simulink model "single_phase_cllc_param"  (R2026a)
settings: Solver=ode23tb  StopTime=param.sim.simlength  FixedStep=tc  MaxStep=param.glb_time.tc
values from neighbouring files (symbols this model uses):
  param = add_template_extras(param, options)    [init_model.m]
libraries: fl_lib x23, nesl_utility x16, lithium_ion_battery x2, full_bridge_ideal_switch x2, full_bridge_mosfet_based_with_thermal_model x2, full_bridge_mosfet_based_with_thermal_model_zvs x2, discrete_time_low_pass_filter x2, single_phase_transformer x1, dab_single_phase_pwm_modulator x1
(part 2 of 2)

== system single_phase_cllc_param/dcdc_cllc_modA/input_current_control/normalization ==
  in : Inport
  1/Ti3 : Gain  Gain=1/param.cllc.hw.Idc_FS  OutDataTypeStr=double  SaturateOnIntegerOverflow=on  ParamDataTypeStr=Inherit: Same as input
  out_pu : Outport
  wires:
  in/1 -> 1/Ti3/1
  1/Ti3/1 -> out_pu/1

== system single_phase_cllc_param/dcdc_cllc_modA/dc//dc with galvanic isolation/full-bridge 1/full-bridge_ideal_switch_based ==
  gate_commands : Inport
  data_measure : Subsystem
  full-bridge_ideal_switch_based : full_bridge_ideal_switch/full-bridge ideal switch based  Rds_on=param.cllc.ideal_switch.Rds_on  Vdon_diode=param.cllc.ideal_switch.Vdon_diode  Rdon_diode=param.cllc.ideal_switch.Rdon_diode  Csnubber=param.cllc.ideal_switch.Csnubber_zvs  Rsnubber=param.cllc.ideal_switch.Rsnubber_zvs  Vth=param.cllc.ideal_switch.Vth
  udc(+) : PMIOPort  Side=Left
  uac(+) : PMIOPort  Port=2  Side=Right
  udc(-) : PMIOPort  Port=3  Side=Left
  uac(-) : PMIOPort  Port=4  Side=Right
  wires:
  full-bridge_ideal_switch_based/1 -> data_measure/1(m)
  gate_commands/1 -> full-bridge_ideal_switch_based/1
  connections:
  udc(+)/RConn1 -- full-bridge_ideal_switch_based/LConn1
  udc(-)/RConn1 -- full-bridge_ideal_switch_based/LConn2
  full-bridge_ideal_switch_based/RConn1 -- uac(+)/RConn1
  uac(-)/RConn1 -- full-bridge_ideal_switch_based/RConn2

== system single_phase_cllc_param/dcdc_cllc_modA/dc//dc with galvanic isolation/full-bridge 1/full-bridge_mosfet_based_with_thermal_model ==
  gate_commands : Inport
  data_measure : Subsystem
  full-bridge_mosfet_based_with_thermal_model : full_bridge_mosfet_based_with_thermal_model/full-bridge mosfet based with thermal model  mass_heatsink_m=param.thermal.weight  specific_heat_m=param.thermal.cp_al  rth_mosfet_HA_m=param.thermal.Rth_mosfet_HA  rth_mosfet_JH_m=param.cllc.mosfet.Rth_mosfet_JH  Rds_on_m=param.cllc.mosfet.Rds_on  Vth_m=param.cllc.mosfet.Vth  Eon_m=param.cllc.mosfet.Eon  Eoff_m=param.cllc.mosfet.Eoff  Voff_sw_loss_m=param.cllc.mosfet.Voff_sw_losses  Ion_sw_loss_m=param.cllc.mosfet.Ion_sw_losses  Vdon_diode_m=param.cllc.mosfet.Vdon_diode  Rdon_diode_m=param.cllc.mosfet.Rds_on  JunctionTermalMass_m=param.cllc.mosfet.JunctionTermalMass  Tambient_m=param.thermal.Tambient  DThs_init_m=param.thermal.DThs_init
  udc(+) : PMIOPort  Side=Left
  uac(+) : PMIOPort  Port=2  Side=Right
  udc(-) : PMIOPort  Port=3  Side=Left
  uac(-) : PMIOPort  Port=4  Side=Right
  wires:
  full-bridge_mosfet_based_with_thermal_model/1 -> data_measure/1(m)
  gate_commands/1 -> full-bridge_mosfet_based_with_thermal_model/1
  connections:
  full-bridge_mosfet_based_with_thermal_model/RConn2 -- uac(-)/RConn1
  full-bridge_mosfet_based_with_thermal_model/LConn1 -- udc(+)/RConn1
  udc(-)/RConn1 -- full-bridge_mosfet_based_with_thermal_model/LConn2
  full-bridge_mosfet_based_with_thermal_model/RConn1 -- uac(+)/RConn1

== system single_phase_cllc_param/dcdc_cllc_modA/dc//dc with galvanic isolation/full-bridge 1/full-bridge_mosfet_based_with_thermal_model_zvs ==
  gate_commands : Inport
  data_measure : Subsystem
  full-bridge_mosfet_based_ with_thermal_model_zvs : full_bridge_mosfet_based_with_thermal_model_zvs/full-bridge_mosfet_based_ with_thermal_model_zvs  mass_heatsink_m=param.thermal.heatsink.no_weight  specific_heat_m=param.thermal.heatsink.cp  rth_mosfet_HA_m=param.thermal.heatsink.Rth_mosfet_HA  rth_mosfet_JH_m=param.cllc.mosfet.Rth_mosfet_JH  Rds_on_m=param.cllc.mosfet.Rds_on  Vth_m=param.cllc.mosfet.Vth  Eon_m=param.cllc.mosfet.Eon  Eoff_m=param.cllc.mosfet.Eoff  Voff_sw_loss_m=param.cllc.mosfet.Voff_sw_losses  Ion_sw_loss_m=param.cllc.mosfet.Ion_sw_losses  Vdon_diode_m=param.cllc.mosfet.Vdon_diode  Rdon_diode_m=param.cllc.mosfet.Rds_on  JunctionTermalMass_m=param.cllc.mosfet.JunctionTermalMass  Tambient_m=param.thermal.Tambient  DThs_init_m=param.thermal.DThs_init  Csnubber_m=param.cllc.mosfet.Csnubber_zvs  Rsnubber_m=param.cllc.mosfet.Rsnubber_zvs
  udc(+) : PMIOPort  Side=Left
  udc(-) : PMIOPort  Port=2  Side=Left
  uac(+) : PMIOPort  Port=3  Side=Right
  uac(-) : PMIOPort  Port=4  Side=Right
  wires:
  full-bridge_mosfet_based_ with_thermal_model_zvs/1 -> data_measure/1(m)
  gate_commands/1 -> full-bridge_mosfet_based_ with_thermal_model_zvs/1
  connections:
  full-bridge_mosfet_based_ with_thermal_model_zvs/LConn2 -- udc(-)/RConn1
  full-bridge_mosfet_based_ with_thermal_model_zvs/LConn1 -- udc(+)/RConn1
  full-bridge_mosfet_based_ with_thermal_model_zvs/RConn2 -- uac(-)/RConn1
  full-bridge_mosfet_based_ with_thermal_model_zvs/RConn1 -- uac(+)/RConn1

== system single_phase_cllc_param/dcdc_cllc_modA/dc//dc with galvanic isolation/full-bridge 2/full-bridge_ideal_switch_based ==
  gate_commands : Inport
  data_measure : Subsystem
  full-bridge_ideal_switch_based : full_bridge_ideal_switch/full-bridge ideal switch based  Rds_on=param.cllc.ideal_switch.Rds_on  Vdon_diode=param.cllc.ideal_switch.Vdon_diode  Rdon_diode=param.cllc.ideal_switch.Rdon_diode  Csnubber=param.cllc.ideal_switch.Csnubber_zvs  Rsnubber=param.cllc.ideal_switch.Rsnubber_zvs  Vth=param.cllc.ideal_switch.Vth
  udc(+) : PMIOPort  Side=Left
  uac(+) : PMIOPort  Port=2  Side=Right
  udc(-) : PMIOPort  Port=3  Side=Left
  uac(-) : PMIOPort  Port=4  Side=Right
  wires:
  full-bridge_ideal_switch_based/1 -> data_measure/1(m)
  gate_commands/1 -> full-bridge_ideal_switch_based/1
  connections:
  udc(+)/RConn1 -- full-bridge_ideal_switch_based/LConn1
  udc(-)/RConn1 -- full-bridge_ideal_switch_based/LConn2
  full-bridge_ideal_switch_based/RConn1 -- uac(+)/RConn1
  uac(-)/RConn1 -- full-bridge_ideal_switch_based/RConn2

== system single_phase_cllc_param/dcdc_cllc_modA/dc//dc with galvanic isolation/full-bridge 2/full-bridge_mosfet_based_with_thermal_model ==
  gate_commands : Inport
  data_measure : Subsystem
  full-bridge_mosfet_based_with_thermal_model : full_bridge_mosfet_based_with_thermal_model/full-bridge mosfet based with thermal model  mass_heatsink_m=param.thermal.weight  specific_heat_m=param.thermal.cp_al  rth_mosfet_HA_m=param.thermal.Rth_mosfet_HA  rth_mosfet_JH_m=param.cllc.mosfet.Rth_mosfet_JH  Rds_on_m=param.cllc.mosfet.Rds_on  Vth_m=param.cllc.mosfet.Vth  Eon_m=param.cllc.mosfet.Eon  Eoff_m=param.cllc.mosfet.Eoff  Voff_sw_loss_m=param.cllc.mosfet.Voff_sw_losses  Ion_sw_loss_m=param.cllc.mosfet.Ion_sw_losses  Vdon_diode_m=param.cllc.mosfet.Vdon_diode  Rdon_diode_m=param.cllc.mosfet.Rds_on  JunctionTermalMass_m=param.cllc.mosfet.JunctionTermalMass  Tambient_m=param.thermal.Tambient  DThs_init_m=param.thermal.DThs_init
  udc(+) : PMIOPort  Side=Left
  uac(+) : PMIOPort  Port=2  Side=Right
  udc(-) : PMIOPort  Port=3  Side=Left
  uac(-) : PMIOPort  Port=4  Side=Right
  wires:
  full-bridge_mosfet_based_with_thermal_model/1 -> data_measure/1(m)
  gate_commands/1 -> full-bridge_mosfet_based_with_thermal_model/1
  connections:
  full-bridge_mosfet_based_with_thermal_model/RConn2 -- uac(-)/RConn1
  full-bridge_mosfet_based_with_thermal_model/LConn1 -- udc(+)/RConn1
  udc(-)/RConn1 -- full-bridge_mosfet_based_with_thermal_model/LConn2
  full-bridge_mosfet_based_with_thermal_model/RConn1 -- uac(+)/RConn1

== system single_phase_cllc_param/dcdc_cllc_modA/dc//dc with galvanic isolation/full-bridge 2/full-bridge_mosfet_based_with_thermal_model_zvs ==
  gate_commands : Inport
  data_measure : Subsystem
  full-bridge_mosfet_based_ with_thermal_model_zvs : full_bridge_mosfet_based_with_thermal_model_zvs/full-bridge_mosfet_based_ with_thermal_model_zvs  mass_heatsink_m=param.thermal.heatsink.no_weight  specific_heat_m=param.thermal.heatsink.cp  rth_mosfet_HA_m=param.thermal.heatsink.Rth_mosfet_HA  rth_mosfet_JH_m=param.cllc.mosfet.Rth_mosfet_JH  Rds_on_m=param.cllc.mosfet.Rds_on  Vth_m=param.cllc.mosfet.Vth  Eon_m=param.cllc.mosfet.Eon  Eoff_m=param.cllc.mosfet.Eoff  Voff_sw_loss_m=param.cllc.mosfet.Voff_sw_losses  Ion_sw_loss_m=param.cllc.mosfet.Ion_sw_losses  Vdon_diode_m=param.cllc.mosfet.Vdon_diode  Rdon_diode_m=param.cllc.mosfet.Rds_on  JunctionTermalMass_m=param.cllc.mosfet.JunctionTermalMass  Tambient_m=param.thermal.Tambient  DThs_init_m=param.thermal.DThs_init  Csnubber_m=param.cllc.mosfet.Csnubber_zvs  Rsnubber_m=param.cllc.mosfet.Rsnubber_zvs
  udc(+) : PMIOPort  Side=Left
  udc(-) : PMIOPort  Port=2  Side=Left
  uac(+) : PMIOPort  Port=3  Side=Right
  uac(-) : PMIOPort  Port=4  Side=Right
  wires:
  full-bridge_mosfet_based_ with_thermal_model_zvs/1 -> data_measure/1(m)
  gate_commands/1 -> full-bridge_mosfet_based_ with_thermal_model_zvs/1
  connections:
  full-bridge_mosfet_based_ with_thermal_model_zvs/LConn2 -- udc(-)/RConn1
  full-bridge_mosfet_based_ with_thermal_model_zvs/LConn1 -- udc(+)/RConn1
  full-bridge_mosfet_based_ with_thermal_model_zvs/RConn2 -- uac(-)/RConn1
  full-bridge_mosfet_based_ with_thermal_model_zvs/RConn1 -- uac(+)/RConn1

== system single_phase_cllc_param/dcdc_cllc_modA/input_current_control/input_current_control/current_control ==
  iout_ref : Inport
  iout : Inport  Port=2
  Sum2 : Sum  Inputs=+-  OutDataTypeStr=double  AccumDataTypeStr=double  SaturateOnIntegerOverflow=on
  iout_ctrl : Subsystem
  ctrli_out : Outport
  wires:
  iout_ctrl/1(phase_shift) -> ctrli_out/1
  iout/1 -> Sum2/2
  iout_ref/1 -> Sum2/1
  Sum2/1 -> iout_ctrl/1(i_tilde)

== system single_phase_cllc_param/dcdc_cllc_modA/dc//dc with galvanic isolation/full-bridge 1/full-bridge_ideal_switch_based/data_measure ==
  m : Inport
  Bus Selector1 : BusSelector  OutputSignals=ideal_switch_current_Q2,ideal_switch_voltage_Q2
  Bus Selector2 : BusSelector  OutputSignals=ideal_switch_current_Q1,ideal_switch_voltage_Q1
  tag scope: idevice_ids_cllc_Q1=global, idevice_ids_cllc_Q2=global, idevice_uds_cllc_Q1=global, idevice_uds_cllc_Q2=global
  wires:
  Bus Selector1/1 -> [idevice_ids_cllc_Q2]  "<ideal_switch_current_Q2>"
  Bus Selector1/2 -> [idevice_uds_cllc_Q2]  "<ideal_switch_voltage_Q2>"
  m/1 -> Bus Selector2/1, Bus Selector1/1
  Bus Selector2/1 -> [idevice_ids_cllc_Q1]  "<ideal_switch_current_Q1>"
  Bus Selector2/2 -> [idevice_uds_cllc_Q1]  "<ideal_switch_voltage_Q1>"

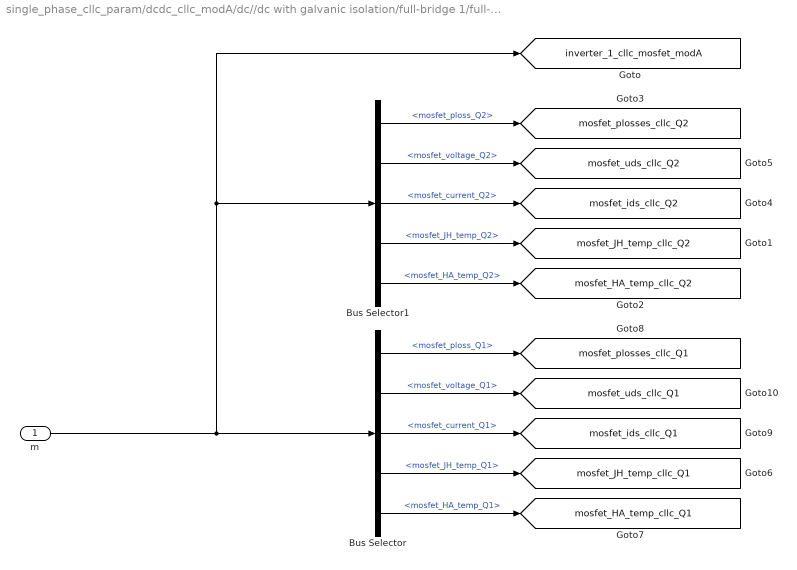
== system single_phase_cllc_param/dcdc_cllc_modA/dc//dc with galvanic isolation/full-bridge 1/full-bridge_mosfet_based_with_thermal_model/data_measure ==
  m : Inport
  Bus Selector : BusSelector  OutputSignals=mosfet_ploss_Q1,mosfet_voltage_Q1,mosfet_current_Q1,mosfet_JH_temp_Q1,mosfet_HA_temp_Q1
  Bus Selector1 : BusSelector  OutputSignals=mosfet_ploss_Q2,mosfet_voltage_Q2,mosfet_current_Q2,mosfet_JH_temp_Q2,mosfet_HA_temp_Q2
  tag scope: inverter_1_cllc_mosfet_modA=global, mosfet_HA_temp_cllc_Q1=global, mosfet_HA_temp_cllc_Q2=global, mosfet_JH_temp_cllc_Q1=global, mosfet_JH_temp_cllc_Q2=global, mosfet_ids_cllc_Q1=global, mosfet_ids_cllc_Q2=global, mosfet_plosses_cllc_Q1=global, mosfet_plosses_cllc_Q2=global, mosfet_uds_cllc_Q1=global, mosfet_uds_cllc_Q2=global
  wires:
  Bus Selector/1 -> [mosfet_plosses_cllc_Q1]  "<mosfet_ploss_Q1>"
  Bus Selector1/3 -> [mosfet_ids_cllc_Q2]  "<mosfet_current_Q2>"
  Bus Selector1/2 -> [mosfet_uds_cllc_Q2]  "<mosfet_voltage_Q2>"
  Bus Selector1/5 -> [mosfet_HA_temp_cllc_Q2]  "<mosfet_HA_temp_Q2>"
  Bus Selector/4 -> [mosfet_JH_temp_cllc_Q1]  "<mosfet_JH_temp_Q1>"
  Bus Selector/5 -> [mosfet_HA_temp_cllc_Q1]  "<mosfet_HA_temp_Q1>"
  Bus Selector1/4 -> [mosfet_JH_temp_cllc_Q2]  "<mosfet_JH_temp_Q2>"
  Bus Selector/3 -> [mosfet_ids_cllc_Q1]  "<mosfet_current_Q1>"
  Bus Selector/2 -> [mosfet_uds_cllc_Q1]  "<mosfet_voltage_Q1>"
  Bus Selector1/1 -> [mosfet_plosses_cllc_Q2]  "<mosfet_ploss_Q2>"
  m/1 -> Bus Selector/1, Bus Selector1/1, [inverter_1_cllc_mosfet_modA]

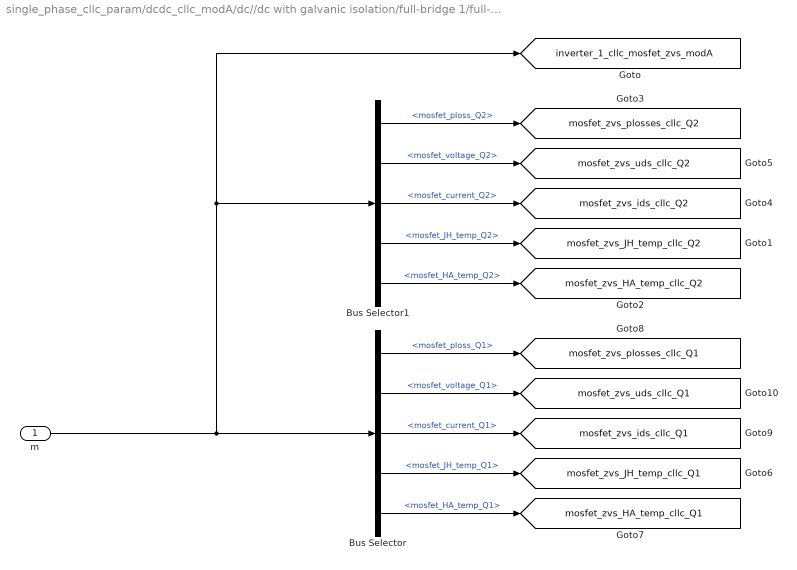
== system single_phase_cllc_param/dcdc_cllc_modA/dc//dc with galvanic isolation/full-bridge 1/full-bridge_mosfet_based_with_thermal_model_zvs/data_measure ==
  m : Inport
  Bus Selector : BusSelector  OutputSignals=mosfet_ploss_Q1,mosfet_voltage_Q1,mosfet_current_Q1,mosfet_JH_temp_Q1,mosfet_HA_temp_Q1
  Bus Selector1 : BusSelector  OutputSignals=mosfet_ploss_Q2,mosfet_voltage_Q2,mosfet_current_Q2,mosfet_JH_temp_Q2,mosfet_HA_temp_Q2
  tag scope: inverter_1_cllc_mosfet_zvs_modA=global, mosfet_zvs_HA_temp_cllc_Q1=global, mosfet_zvs_HA_temp_cllc_Q2=global, mosfet_zvs_JH_temp_cllc_Q1=global, mosfet_zvs_JH_temp_cllc_Q2=global, mosfet_zvs_ids_cllc_Q1=global, mosfet_zvs_ids_cllc_Q2=global, mosfet_zvs_plosses_cllc_Q1=global, mosfet_zvs_plosses_cllc_Q2=global, mosfet_zvs_uds_cllc_Q1=global, mosfet_zvs_uds_cllc_Q2=global
  wires:
  Bus Selector/1 -> [mosfet_zvs_plosses_cllc_Q1]  "<mosfet_ploss_Q1>"
  Bus Selector1/3 -> [mosfet_zvs_ids_cllc_Q2]  "<mosfet_current_Q2>"
  Bus Selector1/2 -> [mosfet_zvs_uds_cllc_Q2]  "<mosfet_voltage_Q2>"
  Bus Selector1/5 -> [mosfet_zvs_HA_temp_cllc_Q2]  "<mosfet_HA_temp_Q2>"
  Bus Selector/4 -> [mosfet_zvs_JH_temp_cllc_Q1]  "<mosfet_JH_temp_Q1>"
  Bus Selector/5 -> [mosfet_zvs_HA_temp_cllc_Q1]  "<mosfet_HA_temp_Q1>"
  Bus Selector1/4 -> [mosfet_zvs_JH_temp_cllc_Q2]  "<mosfet_JH_temp_Q2>"
  Bus Selector/3 -> [mosfet_zvs_ids_cllc_Q1]  "<mosfet_current_Q1>"
  Bus Selector/2 -> [mosfet_zvs_uds_cllc_Q1]  "<mosfet_voltage_Q1>"
  Bus Selector1/1 -> [mosfet_zvs_plosses_cllc_Q2]  "<mosfet_ploss_Q2>"
  m/1 -> Bus Selector/1, Bus Selector1/1, [inverter_1_cllc_mosfet_zvs_modA]

== system single_phase_cllc_param/dcdc_cllc_modA/dc//dc with galvanic isolation/full-bridge 2/full-bridge_ideal_switch_based/data_measure ==
  m : Inport
  Bus Selector1 : BusSelector  OutputSignals=ideal_switch_current_Q2,ideal_switch_voltage_Q2
  Bus Selector2 : BusSelector  OutputSignals=ideal_switch_current_Q1,ideal_switch_voltage_Q1
  tag scope: idevice_ids_cllc_Q5=global, idevice_ids_cllc_Q6=global, idevice_uds_cllc_Q5=global, idevice_uds_cllc_Q6=global
  wires:
  Bus Selector1/1 -> [idevice_ids_cllc_Q6]  "<ideal_switch_current_Q2>"
  Bus Selector1/2 -> [idevice_uds_cllc_Q6]  "<ideal_switch_voltage_Q2>"
  m/1 -> Bus Selector2/1, Bus Selector1/1
  Bus Selector2/1 -> [idevice_ids_cllc_Q5]  "<ideal_switch_current_Q1>"
  Bus Selector2/2 -> [idevice_uds_cllc_Q5]  "<ideal_switch_voltage_Q1>"

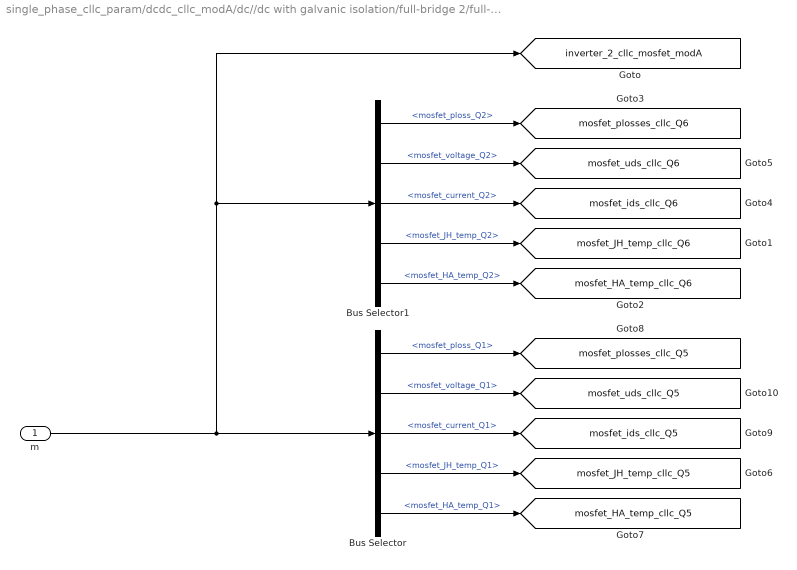
== system single_phase_cllc_param/dcdc_cllc_modA/dc//dc with galvanic isolation/full-bridge 2/full-bridge_mosfet_based_with_thermal_model/data_measure ==
  m : Inport
  Bus Selector : BusSelector  OutputSignals=mosfet_ploss_Q1,mosfet_voltage_Q1,mosfet_current_Q1,mosfet_JH_temp_Q1,mosfet_HA_temp_Q1
  Bus Selector1 : BusSelector  OutputSignals=mosfet_ploss_Q2,mosfet_voltage_Q2,mosfet_current_Q2,mosfet_JH_temp_Q2,mosfet_HA_temp_Q2
  tag scope: inverter_2_cllc_mosfet_modA=global, mosfet_HA_temp_cllc_Q5=global, mosfet_HA_temp_cllc_Q6=global, mosfet_JH_temp_cllc_Q5=global, mosfet_JH_temp_cllc_Q6=global, mosfet_ids_cllc_Q5=global, mosfet_ids_cllc_Q6=global, mosfet_plosses_cllc_Q5=global, mosfet_plosses_cllc_Q6=global, mosfet_uds_cllc_Q5=global, mosfet_uds_cllc_Q6=global
  wires:
  Bus Selector/1 -> [mosfet_plosses_cllc_Q5]  "<mosfet_ploss_Q1>"
  Bus Selector1/3 -> [mosfet_ids_cllc_Q6]  "<mosfet_current_Q2>"
  Bus Selector1/2 -> [mosfet_uds_cllc_Q6]  "<mosfet_voltage_Q2>"
  Bus Selector1/5 -> [mosfet_HA_temp_cllc_Q6]  "<mosfet_HA_temp_Q2>"
  Bus Selector/4 -> [mosfet_JH_temp_cllc_Q5]  "<mosfet_JH_temp_Q1>"
  Bus Selector/5 -> [mosfet_HA_temp_cllc_Q5]  "<mosfet_HA_temp_Q1>"
  Bus Selector1/4 -> [mosfet_JH_temp_cllc_Q6]  "<mosfet_JH_temp_Q2>"
  Bus Selector/3 -> [mosfet_ids_cllc_Q5]  "<mosfet_current_Q1>"
  Bus Selector/2 -> [mosfet_uds_cllc_Q5]  "<mosfet_voltage_Q1>"
  Bus Selector1/1 -> [mosfet_plosses_cllc_Q6]  "<mosfet_ploss_Q2>"
  m/1 -> Bus Selector/1, Bus Selector1/1, [inverter_2_cllc_mosfet_modA]

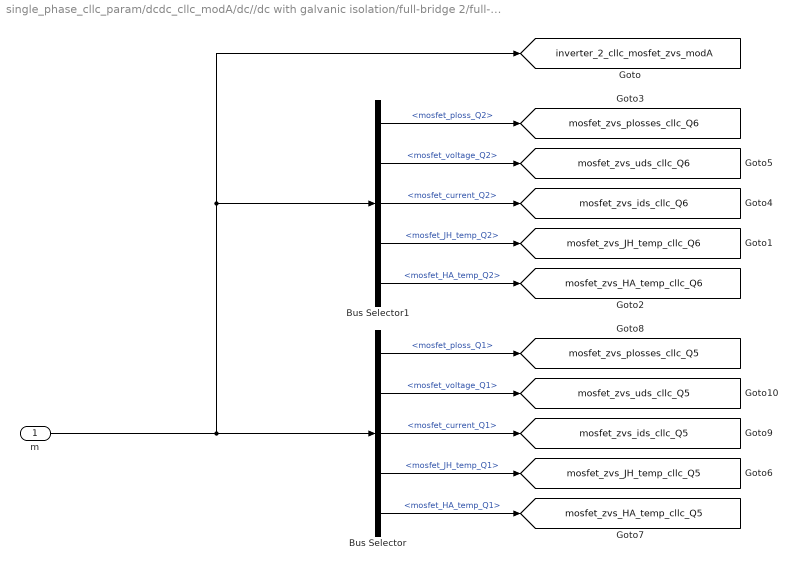
== system single_phase_cllc_param/dcdc_cllc_modA/dc//dc with galvanic isolation/full-bridge 2/full-bridge_mosfet_based_with_thermal_model_zvs/data_measure ==
  m : Inport
  Bus Selector : BusSelector  OutputSignals=mosfet_ploss_Q1,mosfet_voltage_Q1,mosfet_current_Q1,mosfet_JH_temp_Q1,mosfet_HA_temp_Q1
  Bus Selector1 : BusSelector  OutputSignals=mosfet_ploss_Q2,mosfet_voltage_Q2,mosfet_current_Q2,mosfet_JH_temp_Q2,mosfet_HA_temp_Q2
  tag scope: inverter_2_cllc_mosfet_zvs_modA=global, mosfet_zvs_HA_temp_cllc_Q5=global, mosfet_zvs_HA_temp_cllc_Q6=global, mosfet_zvs_JH_temp_cllc_Q5=global, mosfet_zvs_JH_temp_cllc_Q6=global, mosfet_zvs_ids_cllc_Q5=global, mosfet_zvs_ids_cllc_Q6=global, mosfet_zvs_plosses_cllc_Q5=global, mosfet_zvs_plosses_cllc_Q6=global, mosfet_zvs_uds_cllc_Q5=global, mosfet_zvs_uds_cllc_Q6=global
  wires:
  Bus Selector/1 -> [mosfet_zvs_plosses_cllc_Q5]  "<mosfet_ploss_Q1>"
  Bus Selector1/3 -> [mosfet_zvs_ids_cllc_Q6]  "<mosfet_current_Q2>"
  Bus Selector1/2 -> [mosfet_zvs_uds_cllc_Q6]  "<mosfet_voltage_Q2>"
  Bus Selector1/5 -> [mosfet_zvs_HA_temp_cllc_Q6]  "<mosfet_HA_temp_Q2>"
  Bus Selector/4 -> [mosfet_zvs_JH_temp_cllc_Q5]  "<mosfet_JH_temp_Q1>"
  Bus Selector/5 -> [mosfet_zvs_HA_temp_cllc_Q5]  "<mosfet_HA_temp_Q1>"
  Bus Selector1/4 -> [mosfet_zvs_JH_temp_cllc_Q6]  "<mosfet_JH_temp_Q2>"
  Bus Selector/3 -> [mosfet_zvs_ids_cllc_Q5]  "<mosfet_current_Q1>"
  Bus Selector/2 -> [mosfet_zvs_uds_cllc_Q5]  "<mosfet_voltage_Q1>"
  Bus Selector1/1 -> [mosfet_zvs_plosses_cllc_Q6]  "<mosfet_ploss_Q2>"
  m/1 -> Bus Selector/1, Bus Selector1/1, [inverter_2_cllc_mosfet_zvs_modA]

== system single_phase_cllc_param/dcdc_cllc_modA/input_current_control/input_current_control/current_control/iout_ctrl ==
  i_tilde : Inport
  -1 < x < 1 : Saturate  UpperLimit=1  LowerLimit=-1  OutDataTypeStr=double
  1/Ti : Gain  Gain=param.cllc.ctrl.kp_idc  ParamDataTypeStr=double  OutDataTypeStr=double  SaturateOnIntegerOverflow=on
  Sum1 : Sum  Inputs=+++  SaturateOnIntegerOverflow=on
  Sum4 : Sum  Inputs=-+  SaturateOnIntegerOverflow=on
  Unit Delay4 : UnitDelay  SampleTime=-1
  kp2 : Gain  Gain=param.cllc.ctrl.ki_idc*param.glb_time.ts_cllc  ParamDataTypeStr=double  OutDataTypeStr=double  SaturateOnIntegerOverflow=on
  phase_shift : Outport
  wires:
  i_tilde/1 -> kp2/1, 1/Ti/1
  Sum1/1 -> -1 < x < 1/1
  kp2/1 -> Sum1/2
  1/Ti/1 -> Sum1/1, Sum4/1
  Sum4/1 -> Unit Delay4/1
  Unit Delay4/1 -> Sum1/3
  -1 < x < 1/1 -> Sum4/2, phase_shift/1  "phase_shift"
